simulink model "s6_intervento_droni"  (R2025b)
settings: Solver=ode45  StartTime=0.0  StopTime=120  FixedStep=0.002  RelTol=1e-3  EnableMultiTasking=on
libraries: slpidlib x4
settings Model: ExtModeTrigDuration=10000  Creator=sciau  LastModifiedBy=sciau
settings SolverCC: AlgebraicLoopSolver=TrustRegion  PositivePriorityOrder=on
settings DataIOCC: ReturnWorkspaceOutputs=off
settings OptimizationCC: LifeSpan=inf
settings DebuggingCC: UnconnectedInputMsg=warning  UnconnectedOutputMsg=warning  UnconnectedLineMsg=warning  ArithmeticOperatorsInVariantConditions=warning
settings ModelReferenceCC: EnableRefExpFcnMdlSchedulingChecks=on
settings SFSimCC: SimUseLocalCustomCode=off  CustomCodeUndefinedFunction=UseInterfaceOnly
settings RTWCC: SystemTargetFile=quarc_win64.tlc  TemplateMakefile=quarc_default_tmf  RTWUseLocalCustomCode=off  GPUComputeCapability=3.5  Description=QUARC Win64 Target
settings CodeAppCC: StateflowObjectComments=on
settings STFCustomTargetCC: SystemTargetFile=quarc_win64.tlc  TargetPreCompLibLocation=C:\PROGRA~3\QUARC\lib\2016a\win64\release  TargetLangStandard=C99 (ISO)  StopOnOverrun=off  DownloadToTarget=on  Debug=off
settings GRTTargetCC: ExtMode=on  ExtModeMexFile=quarc_comm  TargetPreCompLibLocation=C:\PROGRA~3\QUARC\lib\2016a\win64\release  ParMdlRefBuildCompliant=off  CompOptLevelCompliant=off  CombineOutputUpdateFcns=off  MatFileLogging=off  CPPClassGenCompliant=off  GRTInterface=on  UseToolchainInfoCompliant=off
settings ConfigComp: CovMetricSettings=dswe

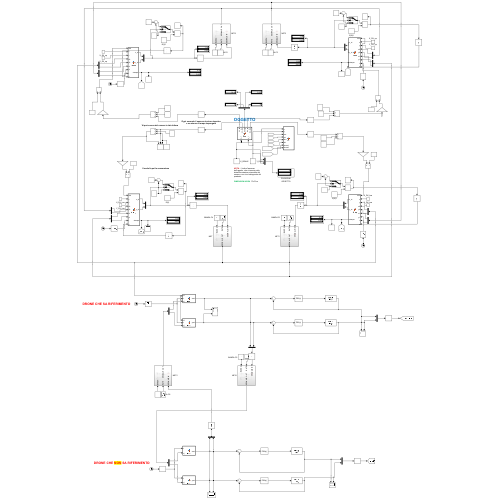
[thumbnail: Simulink's stored preview of the top-level diagram]
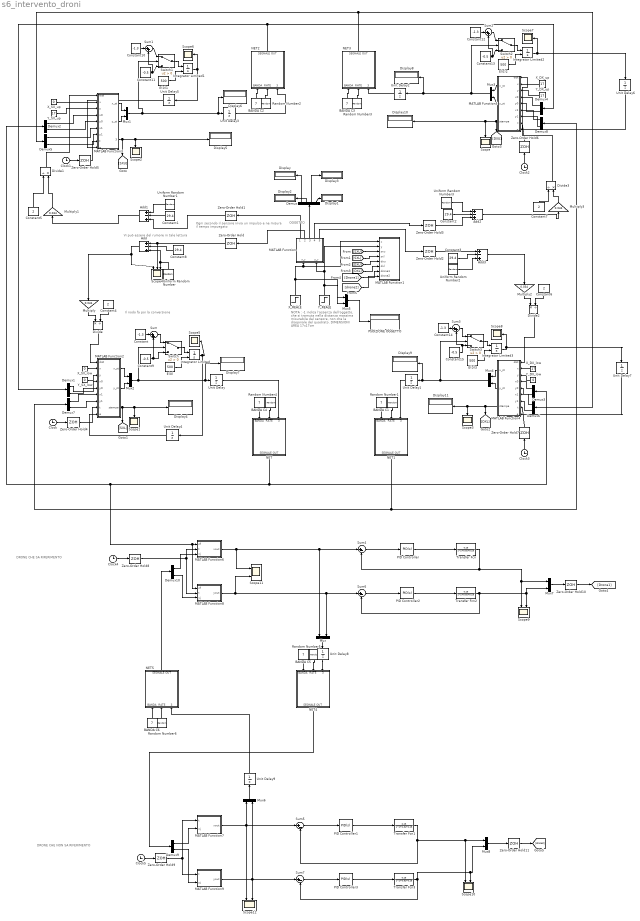
== system s6_intervento_droni ==
  note: DRONE CHE SA RIFERIMENTO
  note: NOTA : -1 indica l'assenza dell'oggetto, che si tramuta nella distanza massima misurabile dal sensore, non che la diagonale del quadrato.
      |
      | DIMENSIONI AREA 17x17cm
  note: OGGETTO
  note: Il nodo fa poi la conversione
  note: Vi può essere del rumore in tale lettura
  note: Ogni secondo il sensore invia un impulso
      | e ne misura il tempo impuegato
  note: DRONE CHE NON SA RIFERIMENTO
  Add{,1..3} (4 alike) : Sum  Inputs=+-+
  BANDA C{1..6} (6 alike) : Constant  Value=7
  Clock{,1..5} (6 alike) : Clock
  Constant{,10,12,14} (4 alike) : Constant  Value=-1.3
  Constant{1..3,8} (4 alike) : Constant  Value=29.4
  Constant{9,11,13,15} (4 alike) : Constant  Value=-0.5
  Constant{4..7} (4 alike) : Constant  Value=2
  Demux : Demux
  Demux{1..10} (10 alike) : Demux  Outputs=2
  Display{,1..11} (12 alike) : Display
  Divide : Product  Inputs=*/
  Divide1 : Product  Inputs=/*
  Divide2 : Product  Inputs=*/
  Divide3 : Product  Inputs=/*
  E(0){,1..3} (4 alike) : Constant  Value=500
  Integrator Limited{,1..3} (4 alike) : Integrator  InitialConditionSource=external  LimitOutput=on  UpperSaturationLimit=500  LowerSaturationLimit=0
  MATLAB Function : MATLAB Function  TreatAsAtomicUnit=on
  MATLAB Function1 : MATLAB Function  TreatAsAtomicUnit=on
  MATLAB Function2 : MATLAB Function  TreatAsAtomicUnit=on
  MATLAB Function3 : MATLAB Function  TreatAsAtomicUnit=on
  MATLAB Function4 : MATLAB Function  TreatAsAtomicUnit=on
  MATLAB Function5 : MATLAB Function  TreatAsAtomicUnit=on
  MATLAB Function6 : MATLAB Function  TreatAsAtomicUnit=on
  MATLAB Function7 : MATLAB Function  TreatAsAtomicUnit=on
  MATLAB Function8 : MATLAB Function  TreatAsAtomicUnit=on
  MATLAB Function9 : MATLAB Function  TreatAsAtomicUnit=on
  Multiply{,1..3} (4 alike) : Gain  Gain=0.034
  Mux{,1..8} (9 alike) : Mux  Inputs=2
  NET : Subsystem
  NET1 : Subsystem
  NET2 : Subsystem
  NET3 : Subsystem
  NET4 : Subsystem
  NET5 : Subsystem
  PID Controller{,1..3} (4 alike) : slpidlib/PID Controller  Controller=PID  Form=Parallel  TimeDomain=Continuous-time  UseExternalTs=off  SampleTime=-1  IntegratorMethod=Forward Euler  FilterMethod=Forward Euler  ControllerParametersSource=internal  P=0.1  I=0.25  UseKiTs=off  D=0  UseExternalDerivativeSource=off  N=100  UseFilter=on  TunerSelectOption=Transfer Function Based (PID Tuner App)  InitialConditionSource=internal  InitialConditionForIntegrator=0  InitialConditionForFilter=0  DifferentiatorICPrevScaledInput=0  ExternalReset=none  TrackingMode=off  Kt=1  LimitOutput=off  SatLimitsSource=internal  UpperSaturationLimit=inf  LowerSaturationLimit=-inf  LinearizeAsGain=on  AntiWindupMode=none  Kb=1  LimitIntegrator=off  UpperIntegratorSaturationLimit=inf  LowerIntegratorSaturationLimit=-inf  POutMin=[]  POutMax=[]  IOutMin=[]  IOutMax=[]  DOutMin=[]  DOutMax=[]  NOutMin=[]  NOutMax=[]  SumOutMin=[]  SumOutMax=[]  SaturationOutMin=[]  SaturationOutMax=[]  PParamMin=[]  PParamMax=[]  IParamMin=[]  IParamMax=[]  DParamMin=[]  DParamMax=[]  NParamMin=[]  NParamMax=[]  KbParamMin=[]  KbParamMax=[]  KtParamMin=[]  KtParamMax=[]  KbOutMin=[]  KbOutMax=[]  KtOutMin=[]  KtOutMax=[]  IntegratorOutMin=[]  IntegratorOutMax=[]  FilterOutMin=[]  FilterOutMax=[]  SumI1OutMin=[]  SumI1OutMax=[]  SumI2OutMin=[]  SumI2OutMax=[]  SumI3OutMin=[]  SumI3OutMax=[]  SumI4OutMin=[]  SumI4OutMax=[]  SumDOutMin=[]  SumDOutMax=[]  DifferentiatorOutMin=[]  DifferentiatorOutMax=[]  FilterDiffOutCoefMin=[]  FilterDiffOutCoefMax=[]  ReciprocalOutMin=[]  ReciprocalOutMax=[]  SumDenOutMin=[]  SumDenOutMax=[]  SumNumOutMin=[]  SumNumOutMax=[]  DivideOutMin=[]  DivideOutMax=[]  UdiffTsProdOutMin=[]  UdiffTsProdOutMax=[]  NTsProdOutMin=[]  NTsProdOutMax=[]  UintegralTsProdOutMin=[]  UintegralTsProdOutMax=[]  UngainTsProdOutMin=[]  UngainTsProdOutMax=[]  ClampingZeroOutDataTypeStr=Inherit: Inherit via back propagation  ClampingZeroOutMin=[]  ClampingZeroOutMax=[]  FilterDenConstantOutDataTypeStr=Inherit: Inherit via back propagation  FilterDenConstantOutMin=[]  FilterDenConstantOutMax=[]  PCopyOutDataTypeStr=Inherit: Inherit via back propagation  PCopyOutMin=[]  PCopyOutMax=[]  NCopyOutDataTypeStr=Inherit: Inherit via back propagation  NCopyOutMin=[]  NCopyOutMax=[]  IntegratorContinuousStateAttributes=''  IntegratorStateMustResolveToSignalObject=off  IntegratorRTWStateStorageClass=Auto  FilterContinuousStateAttributes=''  FilterStateMustResolveToSignalObject=off  FilterRTWStateStorageClass=Auto  ParallelPVariant=InternalParameters  IdealPVariant=Disabled  IVariant=InternalParameters  DVariant=InternalParameters  IntegratorVariant=Continuous  SatVariant=Disabled  AWVariant=Passthrough  PCopyVariant=Disabled  TRVariant=Disabled  FdbkBlocksVariant=Forward  IdealPFdbkVariant=Disabled  SatFdbkVariant=Disabled  DerivativeFilterVariant=ContFilter  NVariant=InternalParameters  NCopyVariant=Disabled  FilterICVariant=InternalICsFilter  IntegratorICVariant=InternalICs  ExternalResetVariant=Disabled  TRSumVariant=Passthrough  SumFdbkVariant=Disabled  SumVariant=Sum_PID  TsampFilterVariant=InternalTs  TsampNgainVariant=Passthrough  TsampIntegralVariant=Disabled_SignalSpec  ExternalSaturationOutDataTypeStr=Inherit: Same as second input  DerivativeSourceVariant=ErrorSignal  PreIntVariant=InternalPreInt
  PSOIZIONE OGGETTO : Display
  Random Number1 : RandomNumber  Mean=6  Variance=6  Seed=2  SampleTime=1
  Random Number2 : RandomNumber  Mean=6  Variance=6  Seed=3  SampleTime=1
  Random Number3 : RandomNumber  Mean=6  Variance=6  Seed=4  SampleTime=1
  Random Number4 : RandomNumber  Mean=6  Variance=6  Seed=1  SampleTime=1
  Random Number5 : RandomNumber  Mean=6  Variance=6  Seed=1  SampleTime=1
  Random Number6 : RandomNumber  Mean=6  Variance=6  Seed=1  SampleTime=1
  Scope{,1..3,5..8} (8 alike) : Scope
      Scope settings: ActiveDisplayYMinimum=-2.5835470868665813  ActiveDisplayYMaximum=13.251923781799233
      Scope1 settings: ActiveDisplayYMinimum=-16.615784549747644  ActiveDisplayYMaximum=28.799818105640938
      Scope2 settings: ActiveDisplayYMinimum=-2.5746656890242572  ActiveDisplayYMaximum=13.171991201218317  DataLoggingVariableName=ScopeData2
      Scope3 settings: ActiveDisplayYMinimum=-2.2144496808462844  ActiveDisplayYMaximum=14.388218564117556  DataLoggingVariableName=ScopeData3
      Scope5 settings: ActiveDisplayYMinimum=258.46250000000026  ActiveDisplayYMaximum=526.8375  DataLoggingVariableName=ScopeData6
      Scope6 settings: ActiveDisplayYMinimum=-3.4505591287330617  ActiveDisplayYMaximum=112.78813117999597  DataLoggingVariableName=ScopeData7
      Scope7 settings: ActiveDisplayYMinimum=-3.4505591287330617  ActiveDisplayYMaximum=112.78813117999597  DataLoggingVariableName=ScopeData8
      Scope8 settings: ActiveDisplayYMinimum=-3.4505591287330617  ActiveDisplayYMaximum=112.78813117999597  DataLoggingVariableName=ScopeData9
  Scope{9..12} (4 alike) : Scope  NumInputPorts=2
      Scope10 settings: ActiveDisplayYMinimum=-4.7307368998935218  ActiveDisplayYMaximum=21.898906574294816  DataLoggingVariableName=ScopeData11
      Scope11 settings: ActiveDisplayYMinimum=-1.4541216702921502  ActiveDisplayYMaximum=13.087095032629353  DataLoggingVariableName=ScopeData12
      Scope12 settings: ActiveDisplayYMinimum=-1.4528995453658229  ActiveDisplayYMaximum=13.076095908292409  DataLoggingVariableName=ScopeData13
      Scope9 settings: ActiveDisplayYMinimum=-4.7307368998935218  ActiveDisplayYMaximum=21.898906574294816  DataLoggingVariableName=ScopeData10
  Scope4 : Scope  NumInputPorts=3
      settings: ActiveDisplayYMinimum=-77.332228841261667  ActiveDisplayYMaximum=1474.6908321791607  DataLoggingVariableName=ScopeData4
  Sum{,1..3} (4 alike) : Sum  Inputs=|++
  Sum{4..7} (4 alike) : Sum  Inputs=|+-
  Switch{,1..3} (4 alike) : Switch  Criteria=u2 > Threshold  SaturateOnIntegerOverflow=off  InputSameDT=off
  Transfer Fcn{,1..3} (4 alike) : TransferFcn  Numerator=[0.25]  Denominator=[1, 0.8, 0.25]
  Uniform Random Number : UniformRandomNumber  Minimum=-17.6  Maximum=17.6  SampleTime=1
  Uniform Random Number1 : UniformRandomNumber  Minimum=-0.3  Maximum=0.3  SampleTime=1
  Uniform Random Number2 : UniformRandomNumber  Minimum=-0.3  Maximum=0.3  SampleTime=1
  Uniform Random Number3 : UniformRandomNumber  Minimum=-0.3  Maximum=0.3  SampleTime=1
  Unit Delay{,1..9} (10 alike) : UnitDelay  SampleTime=-1  HasFrameUpgradeWarning=on
  X_DX_low : Constant  Value=17
  X_DX_up : Constant  Value=17
  X_REALE : Step  Before=-1  After=12  SampleTime=0
  X_SX_low : Constant  Value=0
  X_SX_up : Constant  Value=0
  Y_DX_low : Constant  Value=0
  Y_DX_up : Constant  Value=17
  Y_REALE : Step  Before=-1  After=9  SampleTime=0
  Y_SX_low : Constant  Value=0
  Y_SX_up : Constant  Value=17
  Zero-Order Hold{,1..3} (4 alike) : ZeroOrderHold
  Zero-Order Hold{4..11} (8 alike) : ZeroOrderHold  SampleTime=-1
  wires:
  MATLAB Function4/2(y_st) -> Mux4/2
  MATLAB Function5/3(stampa) -> Display10/1, Scope/1, [DXU]
  Uniform Random Number3/1 -> Add2/1
  NET/1(SEGNALE OUT) -> MATLAB Function8/1(rif), MATLAB Function6/1(rif), Demux2/1, Demux3/1
  Zero-Order Hold3/1 -> Add2/3
  Constant6/1 -> Divide2/2
  Demux5/1 -> MATLAB Function3/6(x1)
  Add/1 -> Multiply/1, Scope4/1
  Random Number3/1 -> NET3/2(RATE)
  Constant2/1 -> Add2/2
  MATLAB Function4/3(stampa) -> [DXL], Scope3/1, Display11/1
  BANDA C3/1 -> NET3/1(BANDA)
  Random Number1/1 -> NET1/2(RATE)
  MATLAB Function3/3(stampa) -> Scope2/1, Display5/1, [SXU]
  Unit Delay3/1 -> NET2/3(SEGNALE IN)
  MATLAB Function/4(dx_up) -> Zero-Order Hold3/1
  NET3/1(SEGNALE OUT) -> Demux6/1, Demux5/1
  Uniform Random Number1/1 -> Add1/1
  MATLAB Function4/1(x_st) -> Mux4/1
  Unit Delay1/1 -> NET1/3(SEGNALE IN)
  Demux7/2 -> MATLAB Function2/7(y1)
  Constant8/1 -> Add/2
  MATLAB Function2/2(y_st) -> Mux2/2
  NET2/1(SEGNALE OUT) -> Demux1/1, Demux4/1
  Unit Delay2/1 -> NET3/3(SEGNALE IN)
  BANDA C2/1 -> NET2/1(BANDA)
  Random Number4/1 -> NET/2(RATE)
  Random Number2/1 -> NET2/2(RATE)
  NET1/1(SEGNALE OUT) -> Demux8/1, Demux7/1
  X_SX_low/1 -> MATLAB Function2/2(x)
  X_REALE/1 -> MATLAB Function/1(x_r), MATLAB Function1/1(x), Mux5/1
  Demux3/1 -> MATLAB Function4/4(x0)
  MATLAB Function5/1(x_st) -> Mux3/1
  Zero-Order Hold/1 -> Scope4/2, Add/1
  Zero-Order Hold4/1 -> MATLAB Function2/8(t)
  MATLAB Function3/1(x_st) -> Mux1/1
  Demux4/2 -> MATLAB Function5/5(y0)
  Demux8/2 -> MATLAB Function5/7(y1)
  [DXU] -> MATLAB Function1/5(dxu)
  Add2/1 -> Multiply3/1
  Demux1/2 -> MATLAB Function2/5(y0)
  Y_SX_up/1 -> MATLAB Function3/3(y)
  BANDA C1/1 -> NET1/1(BANDA)
  MATLAB Function/1(sx_up) -> Zero-Order Hold1/1
  Demux1/1 -> MATLAB Function2/4(x0)
  MATLAB Function/5(dx_low) -> Zero-Order Hold2/1
  Constant7/1 -> Divide3/1
  MATLAB Function2/1(x_st) -> Mux2/1
  Constant4/1 -> Divide/2
  Divide3/1 -> MATLAB Function5/1(dist)
  Multiply/1 -> Divide/1
  Constant5/1 -> Divide1/1
  Uniform Random Number2/1 -> Add3/3
  MATLAB Function/3(debug) -> Demux/1
  Y_DX_up/1 -> MATLAB Function5/3(y)
  MATLAB Function/2(sx_low) -> Zero-Order Hold/1
  X_DX_up/1 -> MATLAB Function5/2(x)
  Y_DX_low/1 -> MATLAB Function4/3(y)
  [SXL] -> MATLAB Function1/4(sxl)
  Demux/2 -> Display2/1
  Uniform Random Number/1 -> Add/3, Scope4/3
  Demux5/2 -> MATLAB Function3/7(y1)
  Divide/1 -> MATLAB Function2/1(dist)
  X_DX_low/1 -> MATLAB Function4/2(x)
  Multiply1/1 -> Divide1/2
  Multiply2/1 -> Divide2/1
  Constant3/1 -> Add3/2
  Demux6/1 -> MATLAB Function4/6(x1)
  Demux/4 -> Display1/1
  Zero-Order Hold1/1 -> Add1/3
  [SXU] -> MATLAB Function1/3(sxu)
  Demux/1 -> Display/1
  Demux/3 -> Display3/1
  Y_REALE/1 -> MATLAB Function/2(y_r), MATLAB Function1/2(y), Mux5/2
  Zero-Order Hold2/1 -> Add3/1
  Add1/1 -> Multiply1/1
  Divide2/1 -> MATLAB Function4/1(dist)
  Demux8/1 -> MATLAB Function5/6(x1)
  Demux3/2 -> MATLAB Function4/5(y0)
  Demux6/2 -> MATLAB Function4/7(y1)
  Multiply3/1 -> Divide3/2
  Demux7/1 -> MATLAB Function2/6(x1)
  MATLAB Function5/2(y_st) -> Mux3/2
  BANDA C4/1 -> NET/1(BANDA)
  Divide1/1 -> MATLAB Function3/1(dist)
  Add3/1 -> Multiply2/1
  Demux2/2 -> MATLAB Function3/5(y0)
  Mux5/1 -> PSOIZIONE OGGETTO/1
  MATLAB Function3/2(y_st) -> Mux1/2
  Constant1/1 -> Add1/2
  Demux2/1 -> MATLAB Function3/4(x0)
  Y_SX_low/1 -> MATLAB Function2/3(y)
  Demux4/1 -> MATLAB Function5/4(x0)
  [DXL] -> MATLAB Function1/6(dxl)
  X_SX_up/1 -> MATLAB Function3/2(x)
  Unit Delay/1 -> NET/3(SEGNALE IN)
  Clock/1 -> Zero-Order Hold4/1
  Clock1/1 -> Zero-Order Hold5/1
  Zero-Order Hold5/1 -> MATLAB Function3/8(t)
  Clock2/1 -> Zero-Order Hold6/1
  Zero-Order Hold6/1 -> MATLAB Function5/8(t)
  Clock3/1 -> Zero-Order Hold7/1
  Zero-Order Hold7/1 -> MATLAB Function4/8(t)
  E(0)/1 -> Integrator Limited/2
  Switch/1 -> Integrator Limited/1
  Constant9/1 -> Sum/2, Switch/3
  Integrator Limited/1 -> Unit Delay4/1, Scope5/1
  Integrator Limited1/1 -> Scope6/1, Unit Delay5/1
  E(0)1/1 -> Integrator Limited1/2
  Switch1/1 -> Integrator Limited1/1
  Integrator Limited2/1 -> Unit Delay6/1, Scope7/1
  E(0)2/1 -> Integrator Limited2/2
  Switch2/1 -> Integrator Limited2/1
  Integrator Limited3/1 -> Unit Delay7/1, Scope8/1
  Mux4/1 -> Switch3/2, Unit Delay1/1, Display9/1
  E(0)3/1 -> Integrator Limited3/2
  Switch3/1 -> Integrator Limited3/1
  Constant/1 -> Sum/1
  Sum/1 -> Switch/1
  Constant10/1 -> Sum1/1
  Sum1/1 -> Switch1/1
  Constant11/1 -> Sum1/2, Switch1/3
  Constant12/1 -> Sum2/1
  Sum2/1 -> Switch2/1
  Constant13/1 -> Sum2/2, Switch2/3
  Constant14/1 -> Sum3/1
  Sum3/1 -> Switch3/1
  Constant15/1 -> Sum3/2, Switch3/3
  Mux2/1 -> Display7/1, Unit Delay/1, Switch/2
  MATLAB Function2/3(stampa) -> Display4/1, Scope1/1, [SXL]
  Mux1/1 -> Display6/1, Unit Delay3/1, Switch1/2
  Mux3/1 -> Display8/1, Unit Delay2/1, Switch2/2
  Unit Delay4/1 -> MATLAB Function2/9(e)
  Unit Delay5/1 -> MATLAB Function3/9(e)
  Unit Delay6/1 -> MATLAB Function5/9(e)
  Unit Delay7/1 -> MATLAB Function4/9(e)
  [Drone1] -> MATLAB Function1/7(drone1)
  [drone2] -> MATLAB Function1/8(drone2)
  Transfer Fcn/1 -> Sum4/2, Mux7/1, Scope9/1
  PID Controller/1 -> Transfer Fcn/1
  Sum4/1 -> PID Controller/1
  MATLAB Function6/1(xout) -> Sum4/1, Mux/1, Scope11/1
  Clock4/1 -> Zero-Order Hold8/1
  Zero-Order Hold8/1 -> MATLAB Function6/2(t), MATLAB Function8/2(t)
  Clock5/1 -> Zero-Order Hold9/1
  Zero-Order Hold9/1 -> MATLAB Function7/1(t), MATLAB Function9/1(t)
  Random Number5/1 -> NET4/2(RATE)
  BANDA C5/1 -> NET4/1(BANDA)
  Random Number6/1 -> NET5/2(RATE)
  BANDA C6/1 -> NET5/1(BANDA)
  MATLAB Function7/1(xout) -> Scope12/1, Mux6/1, Sum5/1
  MATLAB Function9/1(yout) -> Mux6/2, Sum7/1, Scope12/2
  NET4/1(SEGNALE OUT) -> Demux9/1
  NET5/1(SEGNALE OUT) -> Demux10/1
  Demux10/1 -> MATLAB Function6/3(xj)
  Sum5/1 -> PID Controller1/1
  PID Controller1/1 -> Transfer Fcn1/1
  Transfer Fcn1/1 -> Sum5/2, Scope10/1, Mux8/1
  Demux10/2 -> MATLAB Function8/3(yj)
  Sum6/1 -> PID Controller2/1
  PID Controller2/1 -> Transfer Fcn2/1
  Transfer Fcn2/1 -> Sum6/2, Scope9/2, Mux7/2
  MATLAB Function8/1(yout) -> Scope11/2, Sum6/1, Mux/2
  Mux7/1 -> Zero-Order Hold10/1
  Demux9/1 -> MATLAB Function7/2(xj)
  Demux9/2 -> MATLAB Function9/2(yj)
  Transfer Fcn3/1 -> Sum7/2, Mux8/2, Scope10/2
  Sum7/1 -> PID Controller3/1
  PID Controller3/1 -> Transfer Fcn3/1
  Mux8/1 -> Zero-Order Hold11/1
  Unit Delay8/1 -> NET4/3(SEGNALE IN)
  Mux/1 -> Unit Delay8/1
  Unit Delay9/1 -> NET5/3(SEGNALE IN)
  Mux6/1 -> Unit Delay9/1
  Zero-Order Hold10/1 -> [Drone1]
  Zero-Order Hold11/1 -> [drone2]

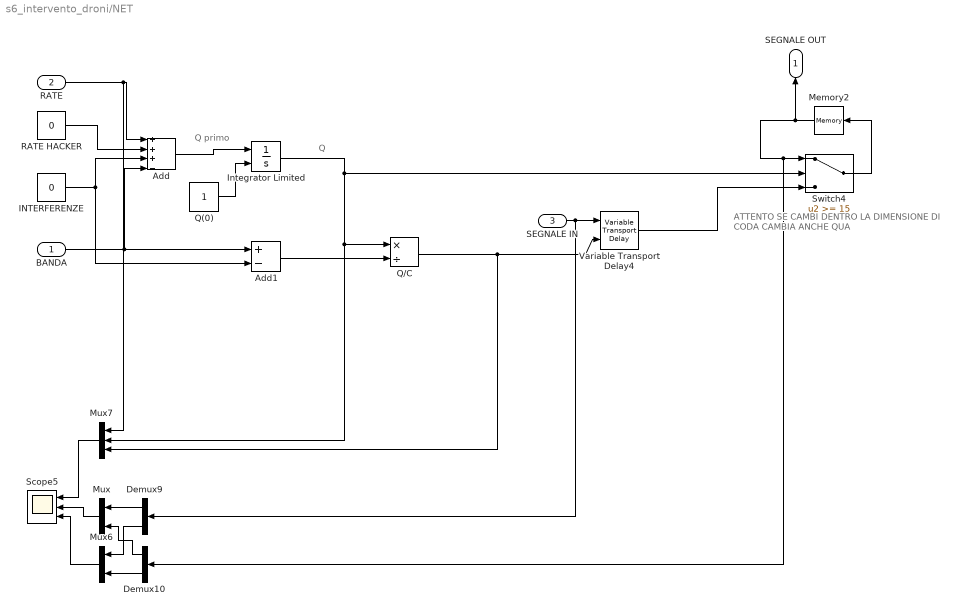
== system s6_intervento_droni/NET ==
  note: Q
  note: Q primo
  note: ATTENTO SE CAMBI
      | DENTRO LA DIMENSIONE DI CODA
      | CAMBIA ANCHE QUA
  BANDA : Inport
  RATE : Inport  Port=2
  SEGNALE IN : Inport  Port=3
  Add : Sum  Inputs=+++-
  Add1 : Sum  Inputs=+-
  Demux10 : Demux  Outputs=2
  Demux9 : Demux  Outputs=2
  INTERFERENZE : Constant  Value=0
  Integrator Limited : Integrator  InitialConditionSource=external  LimitOutput=on  UpperSaturationLimit=15  LowerSaturationLimit=0
  Memory2 : Memory
  Mux : Mux  Inputs=2
  Mux6 : Mux  Inputs=2
  Mux7 : Mux  Inputs=3
  Q(0) : Constant
  Q/C : Product  Inputs=*/
  RATE HACKER : Constant  Value=0
  Scope5 : Scope  NumInputPorts=3
      settings: ActiveDisplayYMinimum=-1  ActiveDisplayYMaximum=1  DataLoggingVariableName=ScopeData5
  Switch4 : Switch  Threshold=15  SaturateOnIntegerOverflow=off  InputSameDT=off
  Variable Transport Delay4 : VariableTransportDelay  MaximumDelay=10  ZeroDelay=on
  SEGNALE OUT : Outport
  wires:
  Add/1 -> Integrator Limited/1
  Q(0)/1 -> Integrator Limited/2
  BANDA/1 -> Add1/1, Add/4
  Add1/1 -> Q/C/2
  INTERFERENZE/1 -> Add/3, Add1/2
  RATE HACKER/1 -> Add/2
  Q/C/1 -> Mux7/3, Variable Transport Delay4/2
  Switch4/1 -> Memory2/1
  Variable Transport Delay4/1 -> Switch4/3
  Memory2/1 -> Switch4/1, Demux10/1, SEGNALE OUT/1
  Integrator Limited/1 -> Mux7/2, Q/C/1, Switch4/2
  SEGNALE IN/1 -> Variable Transport Delay4/1, Demux9/1
  RATE/1 -> Mux7/1, Add/1
  Mux/1 -> Scope5/2
  Mux7/1 -> Scope5/1
  Mux6/1 -> Scope5/3
  Demux9/2 -> Mux6/1
  Demux10/1 -> Mux/2
  Demux9/1 -> Mux/1
  Demux10/2 -> Mux6/2

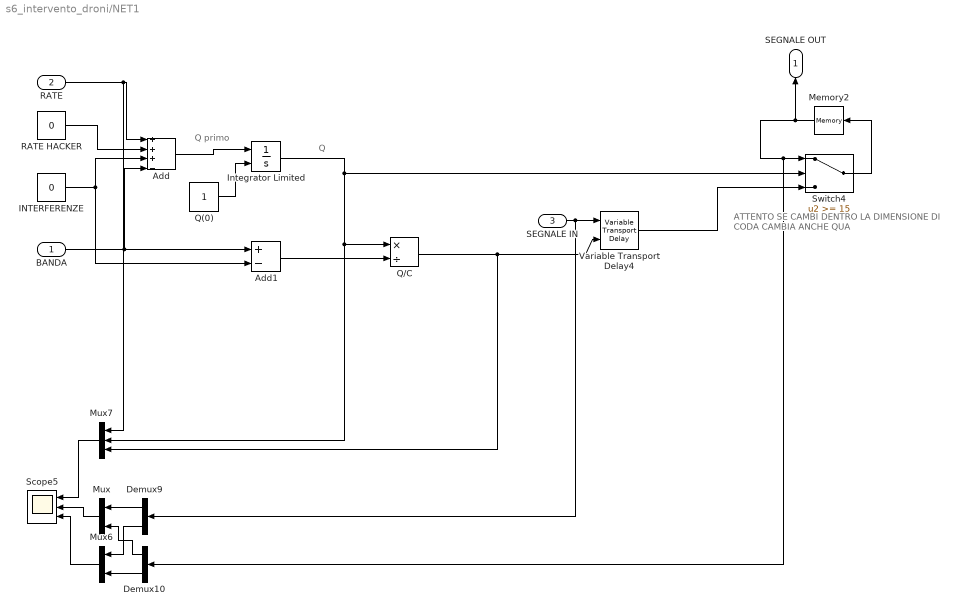
== system s6_intervento_droni/NET1 ==
  note: Q
  note: Q primo
  note: ATTENTO SE CAMBI
      | DENTRO LA DIMENSIONE DI CODA
      | CAMBIA ANCHE QUA
  BANDA : Inport
  RATE : Inport  Port=2
  SEGNALE IN : Inport  Port=3
  Add : Sum  Inputs=+++-
  Add1 : Sum  Inputs=+-
  Demux10 : Demux  Outputs=2
  Demux9 : Demux  Outputs=2
  INTERFERENZE : Constant  Value=0
  Integrator Limited : Integrator  InitialConditionSource=external  LimitOutput=on  UpperSaturationLimit=15  LowerSaturationLimit=0
  Memory2 : Memory
  Mux : Mux  Inputs=2
  Mux6 : Mux  Inputs=2
  Mux7 : Mux  Inputs=3
  Q(0) : Constant
  Q/C : Product  Inputs=*/
  RATE HACKER : Constant  Value=0
  Scope5 : Scope  NumInputPorts=3
      settings: ActiveDisplayYMinimum=-1  ActiveDisplayYMaximum=1  DataLoggingVariableName=ScopeData5
  Switch4 : Switch  Threshold=15  SaturateOnIntegerOverflow=off  InputSameDT=off
  Variable Transport Delay4 : VariableTransportDelay  MaximumDelay=10  ZeroDelay=on
  SEGNALE OUT : Outport
  wires:
  Add/1 -> Integrator Limited/1
  Q(0)/1 -> Integrator Limited/2
  BANDA/1 -> Add1/1, Add/4
  Add1/1 -> Q/C/2
  INTERFERENZE/1 -> Add/3, Add1/2
  RATE HACKER/1 -> Add/2
  Q/C/1 -> Mux7/3, Variable Transport Delay4/2
  Switch4/1 -> Memory2/1
  Variable Transport Delay4/1 -> Switch4/3
  Memory2/1 -> Switch4/1, Demux10/1, SEGNALE OUT/1
  Integrator Limited/1 -> Mux7/2, Q/C/1, Switch4/2
  SEGNALE IN/1 -> Variable Transport Delay4/1, Demux9/1
  RATE/1 -> Mux7/1, Add/1
  Mux/1 -> Scope5/2
  Mux7/1 -> Scope5/1
  Mux6/1 -> Scope5/3
  Demux9/2 -> Mux6/1
  Demux10/1 -> Mux/2
  Demux9/1 -> Mux/1
  Demux10/2 -> Mux6/2

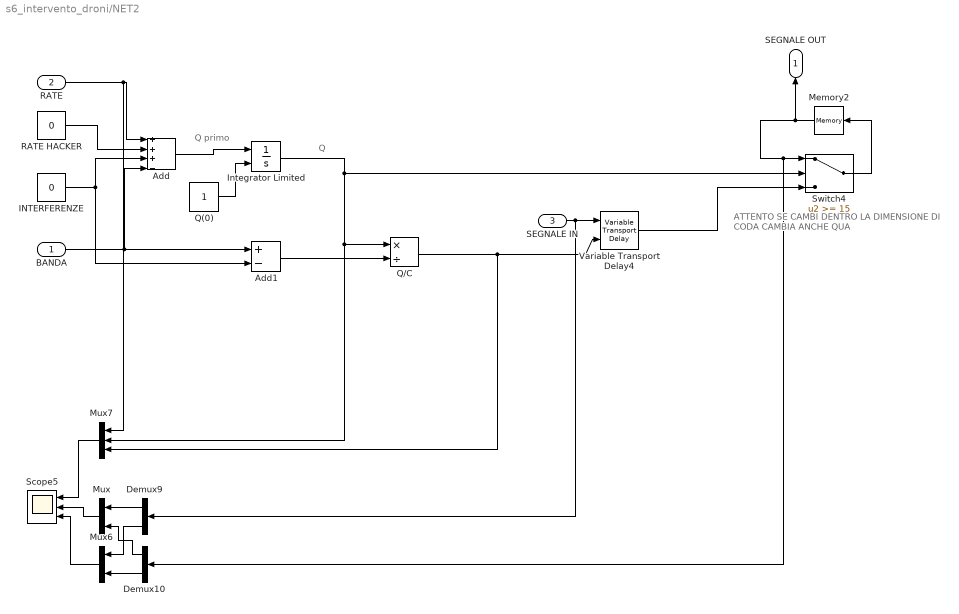
== system s6_intervento_droni/NET2 ==
  note: Q
  note: Q primo
  note: ATTENTO SE CAMBI
      | DENTRO LA DIMENSIONE DI CODA
      | CAMBIA ANCHE QUA
  BANDA : Inport
  RATE : Inport  Port=2
  SEGNALE IN : Inport  Port=3
  Add : Sum  Inputs=+++-
  Add1 : Sum  Inputs=+-
  Demux10 : Demux  Outputs=2
  Demux9 : Demux  Outputs=2
  INTERFERENZE : Constant  Value=0
  Integrator Limited : Integrator  InitialConditionSource=external  LimitOutput=on  UpperSaturationLimit=15  LowerSaturationLimit=0
  Memory2 : Memory
  Mux : Mux  Inputs=2
  Mux6 : Mux  Inputs=2
  Mux7 : Mux  Inputs=3
  Q(0) : Constant
  Q/C : Product  Inputs=*/
  RATE HACKER : Constant  Value=0
  Scope5 : Scope  NumInputPorts=3
      settings: ActiveDisplayYMinimum=-1.8749999999999996  ActiveDisplayYMaximum=16.875  DataLoggingVariableName=ScopeData5
  Switch4 : Switch  Threshold=15  SaturateOnIntegerOverflow=off  InputSameDT=off
  Variable Transport Delay4 : VariableTransportDelay  MaximumDelay=10  ZeroDelay=on
  SEGNALE OUT : Outport
  wires:
  Add/1 -> Integrator Limited/1
  Q(0)/1 -> Integrator Limited/2
  BANDA/1 -> Add1/1, Add/4
  Add1/1 -> Q/C/2
  INTERFERENZE/1 -> Add/3, Add1/2
  RATE HACKER/1 -> Add/2
  Q/C/1 -> Mux7/3, Variable Transport Delay4/2
  Switch4/1 -> Memory2/1
  Variable Transport Delay4/1 -> Switch4/3
  Memory2/1 -> Switch4/1, Demux10/1, SEGNALE OUT/1
  Integrator Limited/1 -> Mux7/2, Q/C/1, Switch4/2
  SEGNALE IN/1 -> Variable Transport Delay4/1, Demux9/1
  RATE/1 -> Mux7/1, Add/1
  Mux/1 -> Scope5/2
  Mux7/1 -> Scope5/1
  Mux6/1 -> Scope5/3
  Demux9/2 -> Mux6/1
  Demux10/1 -> Mux/2
  Demux9/1 -> Mux/1
  Demux10/2 -> Mux6/2

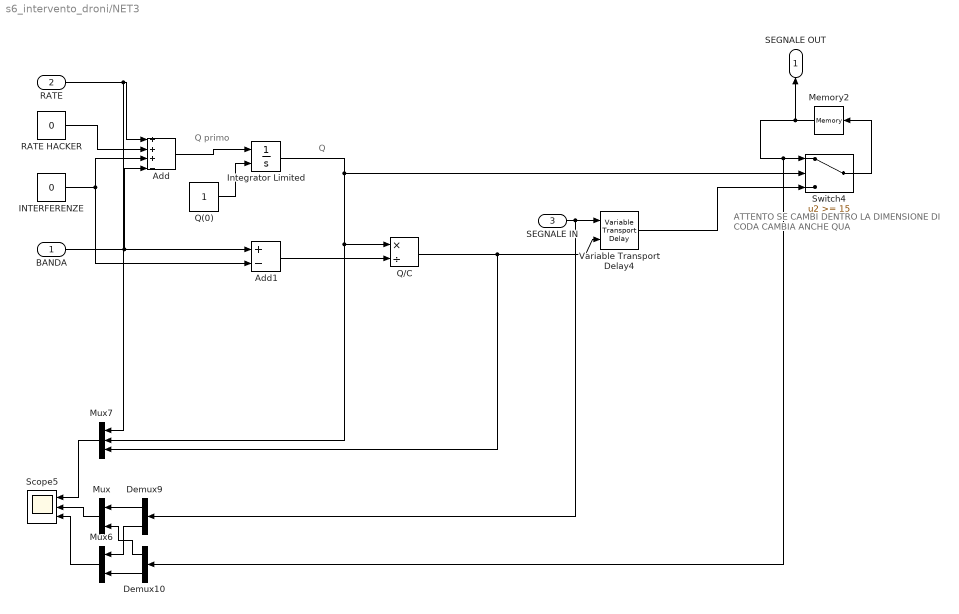
== system s6_intervento_droni/NET3 ==
  note: Q
  note: Q primo
  note: ATTENTO SE CAMBI
      | DENTRO LA DIMENSIONE DI CODA
      | CAMBIA ANCHE QUA
  BANDA : Inport
  RATE : Inport  Port=2
  SEGNALE IN : Inport  Port=3
  Add : Sum  Inputs=+++-
  Add1 : Sum  Inputs=+-
  Demux10 : Demux  Outputs=2
  Demux9 : Demux  Outputs=2
  INTERFERENZE : Constant  Value=0
  Integrator Limited : Integrator  InitialConditionSource=external  LimitOutput=on  UpperSaturationLimit=15  LowerSaturationLimit=0
  Memory2 : Memory
  Mux : Mux  Inputs=2
  Mux6 : Mux  Inputs=2
  Mux7 : Mux  Inputs=3
  Q(0) : Constant
  Q/C : Product  Inputs=*/
  RATE HACKER : Constant  Value=0
  Scope5 : Scope  NumInputPorts=3
      settings: ActiveDisplayYMinimum=-1.8749999999999996  ActiveDisplayYMaximum=16.875  DataLoggingVariableName=ScopeData5
  Switch4 : Switch  Threshold=15  SaturateOnIntegerOverflow=off  InputSameDT=off
  Variable Transport Delay4 : VariableTransportDelay  MaximumDelay=10  ZeroDelay=on
  SEGNALE OUT : Outport
  wires:
  Add/1 -> Integrator Limited/1
  Q(0)/1 -> Integrator Limited/2
  BANDA/1 -> Add1/1, Add/4
  Add1/1 -> Q/C/2
  INTERFERENZE/1 -> Add/3, Add1/2
  RATE HACKER/1 -> Add/2
  Q/C/1 -> Mux7/3, Variable Transport Delay4/2
  Switch4/1 -> Memory2/1
  Variable Transport Delay4/1 -> Switch4/3
  Memory2/1 -> Switch4/1, Demux10/1, SEGNALE OUT/1
  Integrator Limited/1 -> Mux7/2, Q/C/1, Switch4/2
  SEGNALE IN/1 -> Variable Transport Delay4/1, Demux9/1
  RATE/1 -> Mux7/1, Add/1
  Mux/1 -> Scope5/2
  Mux7/1 -> Scope5/1
  Mux6/1 -> Scope5/3
  Demux9/2 -> Mux6/1
  Demux10/1 -> Mux/2
  Demux9/1 -> Mux/1
  Demux10/2 -> Mux6/2

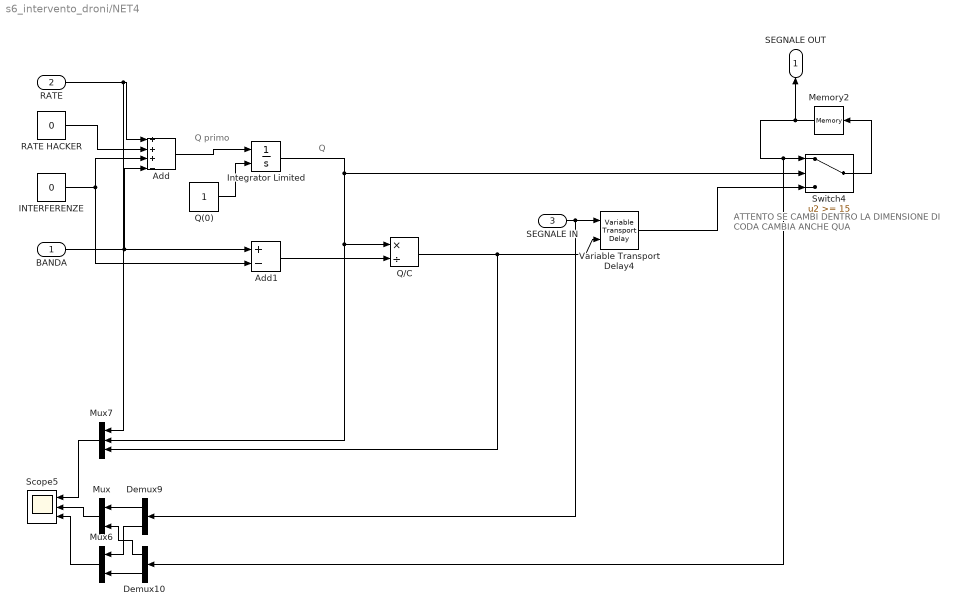
== system s6_intervento_droni/NET4 ==
  note: Q
  note: Q primo
  note: ATTENTO SE CAMBI
      | DENTRO LA DIMENSIONE DI CODA
      | CAMBIA ANCHE QUA
  BANDA : Inport
  RATE : Inport  Port=2
  SEGNALE IN : Inport  Port=3
  Add : Sum  Inputs=+++-
  Add1 : Sum  Inputs=+-
  Demux10 : Demux  Outputs=2
  Demux9 : Demux  Outputs=2
  INTERFERENZE : Constant  Value=0
  Integrator Limited : Integrator  InitialConditionSource=external  LimitOutput=on  UpperSaturationLimit=15  LowerSaturationLimit=0
  Memory2 : Memory
  Mux : Mux  Inputs=2
  Mux6 : Mux  Inputs=2
  Mux7 : Mux  Inputs=3
  Q(0) : Constant
  Q/C : Product  Inputs=*/
  RATE HACKER : Constant  Value=0
  Scope5 : Scope  NumInputPorts=3
      settings: ActiveDisplayYMinimum=-1  ActiveDisplayYMaximum=1  DataLoggingVariableName=ScopeData5
  Switch4 : Switch  Threshold=15  SaturateOnIntegerOverflow=off  InputSameDT=off
  Variable Transport Delay4 : VariableTransportDelay  MaximumDelay=10  ZeroDelay=on
  SEGNALE OUT : Outport
  wires:
  Add/1 -> Integrator Limited/1
  Q(0)/1 -> Integrator Limited/2
  BANDA/1 -> Add1/1, Add/4
  Add1/1 -> Q/C/2
  INTERFERENZE/1 -> Add/3, Add1/2
  RATE HACKER/1 -> Add/2
  Q/C/1 -> Mux7/3, Variable Transport Delay4/2
  Switch4/1 -> Memory2/1
  Variable Transport Delay4/1 -> Switch4/3
  Memory2/1 -> Switch4/1, Demux10/1, SEGNALE OUT/1
  Integrator Limited/1 -> Mux7/2, Q/C/1, Switch4/2
  SEGNALE IN/1 -> Variable Transport Delay4/1, Demux9/1
  RATE/1 -> Mux7/1, Add/1
  Mux/1 -> Scope5/2
  Mux7/1 -> Scope5/1
  Mux6/1 -> Scope5/3
  Demux9/2 -> Mux6/1
  Demux10/1 -> Mux/2
  Demux9/1 -> Mux/1
  Demux10/2 -> Mux6/2

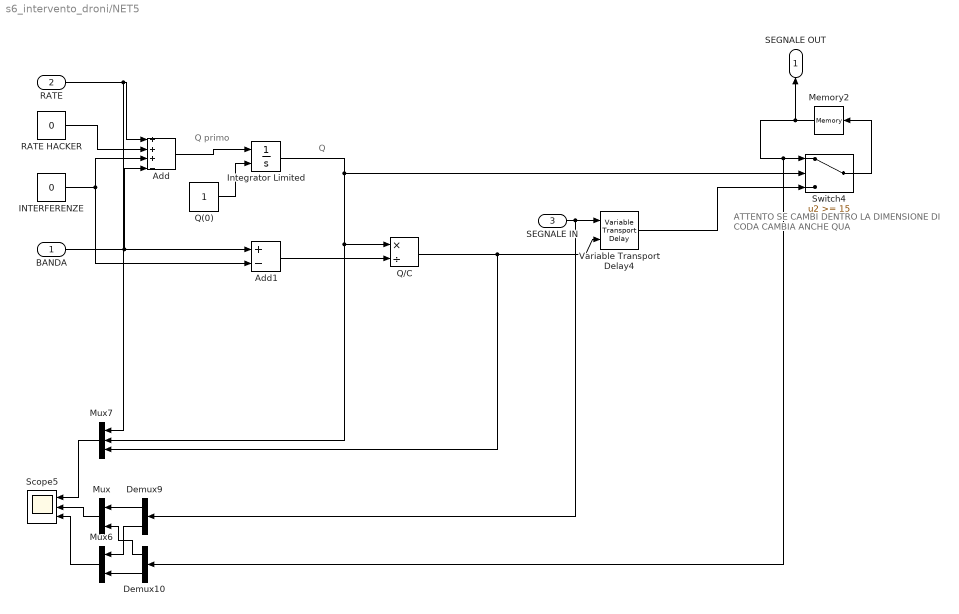
== system s6_intervento_droni/NET5 ==
  note: Q
  note: Q primo
  note: ATTENTO SE CAMBI
      | DENTRO LA DIMENSIONE DI CODA
      | CAMBIA ANCHE QUA
  BANDA : Inport
  RATE : Inport  Port=2
  SEGNALE IN : Inport  Port=3
  Add : Sum  Inputs=+++-
  Add1 : Sum  Inputs=+-
  Demux10 : Demux  Outputs=2
  Demux9 : Demux  Outputs=2
  INTERFERENZE : Constant  Value=0
  Integrator Limited : Integrator  InitialConditionSource=external  LimitOutput=on  UpperSaturationLimit=15  LowerSaturationLimit=0
  Memory2 : Memory
  Mux : Mux  Inputs=2
  Mux6 : Mux  Inputs=2
  Mux7 : Mux  Inputs=3
  Q(0) : Constant
  Q/C : Product  Inputs=*/
  RATE HACKER : Constant  Value=0
  Scope5 : Scope  NumInputPorts=3
      settings: ActiveDisplayYMinimum=-1  ActiveDisplayYMaximum=1  DataLoggingVariableName=ScopeData5
  Switch4 : Switch  Threshold=15  SaturateOnIntegerOverflow=off  InputSameDT=off
  Variable Transport Delay4 : VariableTransportDelay  MaximumDelay=10  ZeroDelay=on
  SEGNALE OUT : Outport
  wires:
  Add/1 -> Integrator Limited/1
  Q(0)/1 -> Integrator Limited/2
  BANDA/1 -> Add1/1, Add/4
  Add1/1 -> Q/C/2
  INTERFERENZE/1 -> Add/3, Add1/2
  RATE HACKER/1 -> Add/2
  Q/C/1 -> Mux7/3, Variable Transport Delay4/2
  Switch4/1 -> Memory2/1
  Variable Transport Delay4/1 -> Switch4/3
  Memory2/1 -> Switch4/1, Demux10/1, SEGNALE OUT/1
  Integrator Limited/1 -> Mux7/2, Q/C/1, Switch4/2
  SEGNALE IN/1 -> Variable Transport Delay4/1, Demux9/1
  RATE/1 -> Mux7/1, Add/1
  Mux/1 -> Scope5/2
  Mux7/1 -> Scope5/1
  Mux6/1 -> Scope5/3
  Demux9/2 -> Mux6/1
  Demux10/1 -> Mux/2
  Demux9/1 -> Mux/1
  Demux10/2 -> Mux6/2

== matlab function s6_intervento_droni/MATLAB Function6 ==
  data: rif input; xout output; t input; xj input
function xout  = assex(rif, t, xj)

   

    persistent x
    persistent riferimento;

    if isempty(x) && isempty(riferimento)
        x=0;
        riferimento=0;
    end

    if t==80
        riferimento=rif(1);
    end
   
    if t>80
        x=x-1*0.5*(x-xj)-1*0.5*(x-riferimento);
        xout=x;
    else
        xout=0;
    end

end

== matlab function s6_intervento_droni/MATLAB Function7 ==
  data: xout output; t input; xj input
function xout  = assex(t, xj) 

    persistent x

    if isempty(x)
        x=0;
    end
   
    if t>80
        x=x-1*0.5*(x-xj);
        xout=x;
    else
        xout=0;
    end
end

== matlab function s6_intervento_droni/MATLAB Function8 ==
  data: rif input; yout output; t input; yj input
function yout  = assey(rif, t, yj)

   

    persistent y
    persistent riferimento;

    if isempty(y) && isempty(riferimento)
        y=0;
        riferimento=0;
    end

    if t==80
        riferimento=rif(2);
    end
   
    if t>80
        y=y-1*0.5*(y-yj)-1*0.5*(y-riferimento);
        yout=y;
    else
        yout=0;
    end

end

== matlab function s6_intervento_droni/MATLAB Function9 ==
  data: yout output; t input; yj input
function yout  = assey(t, yj)

   

    persistent y


    if isempty(y)
        y=0;
    end

   
    if t>80
        y=y-1*0.5*(y-yj);
        yout=y;
    else
        yout=0;
    end

end

== matlab function s6_intervento_droni/MATLAB Function1 ==
  data: x input; y input; sxu input; sxl input; dxu input; dxl input; drone1 input; drone2 input
function dis(x,y,sxu,sxl,dxu,dxl, drone1, drone2)

    % Mantieni il grafico attivo tra le chiamate
    persistent firstRun
    if isempty(firstRun)
        firstRun = true;
    end

    % --- Disegno iniziale del quadrato (solo la prima volta) ---
    if firstRun
        clf;
        axis equal;
        grid on;
        hold on;

        % Centro del quadrato
        cx = 8.5;
        cy = 8.5;
        L = 17;

        % Vertici del quadrato
        X = [cx-L/2, cx+L/2, cx+L/2, cx-L/2, cx-L/2];
        Y = [cy-L/2, cy-L/2, cy+L/2, cy+L/2, cy-L/2];

        plot(X, Y, 'b-', 'LineWidth', 2);
        firstRun = false;
    end

    % --- Disegno dei punti SOLO quando cambiano valore ---
    if x > -1 && y > -1
        plot(x, y, 'ro', 'MarkerSize', 10, 'LineWidth', 2);
        plot(sxu(1), sxu(2), 'go', 'MarkerSize', 3, 'LineWidth', 2);
        plot(sxl(1), sxl(2), 'mo', 'MarkerSize', 3, 'LineWidth', 2);
        plot(dxu(1), dxu(2), 'co', 'MarkerSize', 3, 'LineWidth', 2);
        plot(dxl(1), dxl(2), 'yo', 'MarkerSize', 3, 'LineWidth', 2);

        plot(drone1(1), drone2(2), 'bo', 'MarkerSize', 6, 'LineWidth', 2);
        plot(drone2(1), drone2(2), 'wo', 'MarkerSize', 6, 'LineWidth', 2);
    end


end

== matlab function s6_intervento_droni/MATLAB Function ==
  data: x_r input; sx_up output; y_r input; sx_low output; debug output; dx_up output; dx_low output
function [sx_up, sx_low, debug, dx_up, dx_low]= fcn(x_r, y_r)

idle_dist=22;
idle_time=(idle_dist*2)/0.034;

if x_r==-1 && y_r==-1
        sx_up=idle_time;
        sx_low=idle_time;
        dx_low=idle_time;
        dx_up=idle_time;

        debug=[idle_dist,idle_dist,idle_dist,idle_dist];
else
    
    debug=[-1,-1,-1,-1];

    %sensore in (0,0)
    %0=a*0+q->q=0
    %y_r=a*x_r+0
    
    a=y_r/x_r;
    %vedo se è nel range di coefficienti angolari per cui il punto è nel
    %cono di visione

    if a>tand(30) && a<tand(60)
        cm=sqrt((0-x_r)^2+(0-y_r)^2);
        sx_low=(cm*2)/0.034;
        debug(2)=cm;
    else
        sx_low=idle_time;
        debug(2)=idle_dist;
    end
    
    

    %sensore in (17,17)
    %17=a*17+q->q=17-a*17
    %y_r=a*x_r+q=a*x_r+17-a*17
    
    a=(y_r-17)/(x_r-17);
    %vedo se è nel range di coefficienti angolari per cui il punto è nel
    %cono di visione

    if a>tand(30) && a<tand(60)
        cm=sqrt((17-x_r)^2+(17-y_r)^2);
        dx_up=(cm*2)/0.034;
        debug(3)=cm;
    else
        dx_up=idle_time;
        debug(3)=idle_dist;
    end

    

    %sensore in (0,17)
    %17=a*0+q->q=17
    %y_r=a*x_r+q=a*x_r+17
    
    a=(y_r-17)/(x_r);
    %vedo se è nel range di coefficienti angolari per cui il punto è nel
    %cono di visione

    if a>tand(120) && a<tand(150)
        cm=sqrt((0-x_r)^2+(17-y_r)^2);
        sx_up=(cm*2)/0.034;
        debug(1)=cm;
    else
        sx_up=idle_time;
        debug(1)=idle_dist;
    end

    

    %sensore in (17,0)
    %0=a*17+q->q=-a17
    %y_r=a*x_r+q=a*x_r-a17
    
    a=(y_r)/(x_r-17);
    %vedo se è nel range di coefficienti angolari per cui il punto è nel
    %cono di visione

    if a>tand(120) && a<tand(150)
        cm=sqrt((17-x_r)^2+(0-y_r)^2);
        dx_low=(cm*2)/0.034;
        debug(4)=cm;
    else
        dx_low=idle_time;
        debug(4)=idle_dist;
    end

    

end

end

== matlab function s6_intervento_droni/MATLAB Function2 ==
  data: dist input; x input; y input; x_st output; y_st output; x0 input; y0 input; x1 input; y1 input; stampa output; t input; e input
function [x_st, y_st,stampa] = triang(dist,x,y, x0, y0,x1,y1,t,e)

   

    persistent xst
    persistent yst;

    if isempty(xst) && isempty(yst)
        xst=0.1;
        yst=0.1;
    end

   
    if e>0
        if t<=40
            if dist<=20  
                x_st=xst;
                y_st=yst;
                lo_vedo=1;
            else
                x_st=-1;
                y_st=-1;
                lo_vedo=0;
            end
        
            x_medio=xst;
            y_medio=yst;
            n=1;
        
            if x0~=-1
                x_medio=x_medio+x0;
                y_medio=y_medio+y0;
                n=n+1;
            end
            if x1~=-1
                x_medio=x_medio+x1;
                y_medio=y_medio+y1;
                n=n+1;
            end
        
            x_medio=x_medio/n;
            y_medio=y_medio/n;
        
            if lo_vedo==1
                rx = x_medio-x;
                ry = y_medio-y;
                r=sqrt(rx*rx+ry*ry);
                error=r-dist;
            
                ux=rx/r;
                uy=ry/r;
            
                xst = x_medio - 0.5 * error * ux;
                yst = y_medio - 0.5 * error * uy;
            else
                xst = x_medio;
                yst = y_medio;
            end
        
            stampa=[xst,yst];
        else
    
    
            if x0~=-1
                xst=xst-0.5*1*(xst-x0);
                yst=yst-0.5*1*(yst-y0);
            end
            if x1~=-1
                xst=xst-0.5*1*(xst-x1);     
                yst=yst-0.5*1*(yst-y1);
            end
    
    
            x_st=xst;
            y_st=yst;
    
            stampa=[xst,yst];
        end
    else
        x_st=-1;
        y_st=-1;
        stampa=[-1,-1];
    end

end

== matlab function s6_intervento_droni/MATLAB Function3 ==
  data: dist input; x input; y input; x_st output; y_st output; x0 input; y0 input; x1 input; y1 input; stampa output; t input; e input
function [x_st, y_st,stampa] = triang(dist,x,y, x0, y0,x1,y1,t,e)

   

    persistent xst
    persistent yst;

    if isempty(xst) && isempty(yst)
        xst=0.1;
        yst=0.1;
    end

   
    if e>0
        if t<=40
            if dist<=20  
                x_st=xst;
                y_st=yst;
                lo_vedo=1;
            else
                x_st=-1;
                y_st=-1;
                lo_vedo=0;
            end
        
            x_medio=xst;
            y_medio=yst;
            n=1;
        
            if x0~=-1
                x_medio=x_medio+x0;
                y_medio=y_medio+y0;
                n=n+1;
            end
            if x1~=-1
                x_medio=x_medio+x1;
                y_medio=y_medio+y1;
                n=n+1;
            end
        
            x_medio=x_medio/n;
            y_medio=y_medio/n;
        
            if lo_vedo==1
                rx = x_medio-x;
                ry = y_medio-y;
                r=sqrt(rx*rx+ry*ry);
                error=r-dist;
            
                ux=rx/r;
                uy=ry/r;
            
                xst = x_medio - 0.5 * error * ux;
                yst = y_medio - 0.5 * error * uy;
            else
                xst = x_medio;
                yst = y_medio;
            end
        
            stampa=[xst,yst];
        else
    
    
            if x0~=-1
                xst=xst-0.5*1*(xst-x0);
                yst=yst-0.5*1*(yst-y0);
            end
            if x1~=-1
                xst=xst-0.5*1*(xst-x1);     
                yst=yst-0.5*1*(yst-y1);
            end
    
    
            x_st=xst;
            y_st=yst;
    
            stampa=[xst,yst];
        end
    else
        x_st=-1;
        y_st=-1;
        stampa=[-1,-1];
    end

end

== matlab function s6_intervento_droni/MATLAB Function4 ==
  data: dist input; x input; y input; x_st output; y_st output; x0 input; y0 input; x1 input; y1 input; stampa output; t input; e input
function [x_st, y_st,stampa] = triang(dist,x,y, x0, y0,x1,y1,t,e)

   

    persistent xst
    persistent yst;

    if isempty(xst) && isempty(yst)
        xst=0.1;
        yst=0.1;
    end

   
    if e>0
        if t<=40
            if dist<=20  
                x_st=xst;
                y_st=yst;
                lo_vedo=1;
            else
                x_st=-1;
                y_st=-1;
                lo_vedo=0;
            end
        
            x_medio=xst;
            y_medio=yst;
            n=1;
        
            if x0~=-1
                x_medio=x_medio+x0;
                y_medio=y_medio+y0;
                n=n+1;
            end
            if x1~=-1
                x_medio=x_medio+x1;
                y_medio=y_medio+y1;
                n=n+1;
            end
        
            x_medio=x_medio/n;
            y_medio=y_medio/n;
        
            if lo_vedo==1
                rx = x_medio-x;
                ry = y_medio-y;
                r=sqrt(rx*rx+ry*ry);
                error=r-dist;
            
                ux=rx/r;
                uy=ry/r;
            
                xst = x_medio - 0.5 * error * ux;
                yst = y_medio - 0.5 * error * uy;
            else
                xst = x_medio;
                yst = y_medio;
            end
        
            stampa=[xst,yst];
        else
    
    
            if x0~=-1
                xst=xst-0.5*1*(xst-x0);
                yst=yst-0.5*1*(yst-y0);
            end
            if x1~=-1
                xst=xst-0.5*1*(xst-x1);     
                yst=yst-0.5*1*(yst-y1);
            end
    
    
            x_st=xst;
            y_st=yst;
    
            stampa=[xst,yst];
        end
    else
        x_st=-1;
        y_st=-1;
        stampa=[-1,-1];
    end

end

== matlab function s6_intervento_droni/MATLAB Function5 ==
  data: dist input; x input; y input; x_st output; y_st output; x0 input; y0 input; x1 input; y1 input; stampa output; t input; e input
function [x_st, y_st,stampa] = triang(dist,x,y, x0, y0,x1,y1,t,e)

   

    persistent xst
    persistent yst;

    if isempty(xst) && isempty(yst)
        xst=0.1;
        yst=0.1;
    end

   
    if e>0
        if t<=40
            if dist<=20  
                x_st=xst;
                y_st=yst;
                lo_vedo=1;
            else
                x_st=-1;
                y_st=-1;
                lo_vedo=0;
            end
        
            x_medio=xst;
            y_medio=yst;
            n=1;
        
            if x0~=-1
                x_medio=x_medio+x0;
                y_medio=y_medio+y0;
                n=n+1;
            end
            if x1~=-1
                x_medio=x_medio+x1;
                y_medio=y_medio+y1;
                n=n+1;
            end
        
            x_medio=x_medio/n;
            y_medio=y_medio/n;
        
            if lo_vedo==1
                rx = x_medio-x;
                ry = y_medio-y;
                r=sqrt(rx*rx+ry*ry);
                error=r-dist;
            
                ux=rx/r;
                uy=ry/r;
            
                xst = x_medio - 0.5 * error * ux;
                yst = y_medio - 0.5 * error * uy;
            else
                xst = x_medio;
                yst = y_medio;
            end
        
            stampa=[xst,yst];
        else
    
    
            if x0~=-1
                xst=xst-0.5*1*(xst-x0);
                yst=yst-0.5*1*(yst-y0);
            end
            if x1~=-1
                xst=xst-0.5*1*(xst-x1);     
                yst=yst-0.5*1*(yst-y1);
            end
    
    
            x_st=xst;
            y_st=yst;
    
            stampa=[xst,yst];
        end
    else
        x_st=-1;
        y_st=-1;
        stampa=[-1,-1];
    end

end
